simulink model "BLDCSpeedControl_EV_Layout_v2_backup_before_step3"  (R2024b)
settings: Solver=ode23t  StartTime=0.0  StopTime=0.3  FixedStep=Ts  MaxStep=5e-4  RelTol=1e-3  EnableMultiTasking=on
PreLoadFcn:
  | BLDCSpeedControlData;
PostLoadFcn:
  | % [EV_DAQ_V7_HOOK]
  | try; EV_DAQ_Builder_V7('LoadStop'); catch; end
InitFcn:
  | % [EV_DAQ_V7_HOOK]
  | try; EV_DAQ_Builder_V7('Overrides'); catch ME__daq; fprintf('[DAQ] Overrides error: %s\n', ME__daq.message); end
StartFcn:
  | % [EV_DAQ_V7_HOOK]
  | try; EV_DAQ_Builder_V7('AutoInit'); catch ME__daq; fprintf('[DAQ] Auto-init error: %s\n', ME__daq.message); end
StopFcn:
  | % [EV_DAQ_V7_HOOK]
  | try; EV_DAQ_Builder_V7('PostProcess'); catch ME__daq; fprintf('[DAQ] Post-process error: %s\n', ME__daq.message); end
undefined symbols (not defined in the file): battery_builder_rtmsupport, cells_parallel, cells_series, DiscIntNeverNeededParam, Emax, Emax_thr, emf_max_ev, gcbh, I_cont, I_peak, Ke_ph, Kii, Kiv, Kiw, Kpi, Kpv, Kpw, load_scale, p, r_wheel, rpm_ramp, rpm_ref, T_Ifilt, Ts, Tsc, Vdc, Vlim_min, wheel_mass
libraries: nesl_utility x17, fl_lib x17, ee_lib x6, eeDiscretePi x2, Batteries2_lib x1, SignalEditorBlockLib x1, eePwmGenerator x1, eeGeneralControl x1
(part 2 of 2)

== system BLDCSpeedControl_EV_Layout_v2_backup_before_step3/Speed//RPM Controller/Sign ==
  u : Inport
  Constant2 : Constant
  Constant3 : Constant  Value=-1
  Switch : Switch  SaturateOnIntegerOverflow=off  InputSameDT=off
  y : Outport
  wires:
  Constant3/1 -> Switch/3
  Constant2/1 -> Switch/1
  u/1 -> Switch/2
  Switch/1 -> y/1

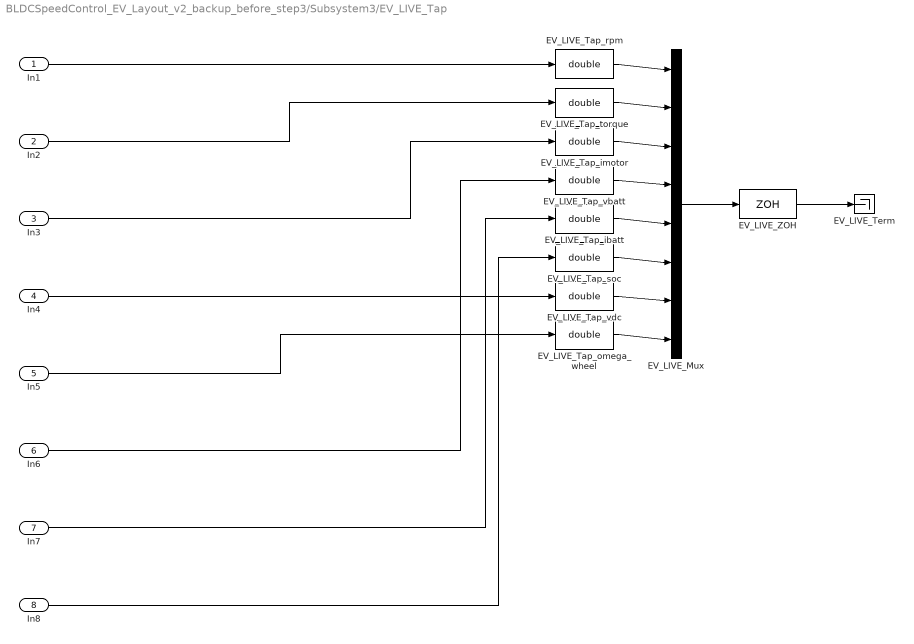
== system BLDCSpeedControl_EV_Layout_v2_backup_before_step3/Subsystem3/EV_LIVE_Tap ==
  In1 : Inport
  In2 : Inport  Port=2
  In3 : Inport  Port=3
  In4 : Inport  Port=4
  In5 : Inport  Port=5
  In6 : Inport  Port=6
  In7 : Inport  Port=7
  In8 : Inport  Port=8
  EV_LIVE_Mux : Mux  Inputs=8
  EV_LIVE_Tap_ibatt : DataTypeConversion  OutDataTypeStr=double
  EV_LIVE_Tap_imotor : DataTypeConversion  OutDataTypeStr=double
  EV_LIVE_Tap_omega_wheel : DataTypeConversion  OutDataTypeStr=double
  EV_LIVE_Tap_rpm : DataTypeConversion  OutDataTypeStr=double
  EV_LIVE_Tap_soc : DataTypeConversion  OutDataTypeStr=double
  EV_LIVE_Tap_torque : DataTypeConversion  OutDataTypeStr=double
  EV_LIVE_Tap_vbatt : DataTypeConversion  OutDataTypeStr=double
  EV_LIVE_Tap_vdc : DataTypeConversion  OutDataTypeStr=double
  EV_LIVE_Term : Terminator
  EV_LIVE_ZOH : ZeroOrderHold  SampleTime=0.1
  wires:
  EV_LIVE_Mux/1 -> EV_LIVE_ZOH/1
  EV_LIVE_Tap_rpm/1 -> EV_LIVE_Mux/1
  In5/1 -> EV_LIVE_Tap_omega_wheel/1
  EV_LIVE_Tap_imotor/1 -> EV_LIVE_Mux/3
  EV_LIVE_ZOH/1 -> EV_LIVE_Term/1
  EV_LIVE_Tap_torque/1 -> EV_LIVE_Mux/2
  EV_LIVE_Tap_ibatt/1 -> EV_LIVE_Mux/5
  In6/1 -> EV_LIVE_Tap_vbatt/1
  EV_LIVE_Tap_vbatt/1 -> EV_LIVE_Mux/4
  EV_LIVE_Tap_omega_wheel/1 -> EV_LIVE_Mux/8
  EV_LIVE_Tap_soc/1 -> EV_LIVE_Mux/6
  EV_LIVE_Tap_vdc/1 -> EV_LIVE_Mux/7
  In8/1 -> EV_LIVE_Tap_soc/1
  In1/1 -> EV_LIVE_Tap_rpm/1
  In2/1 -> EV_LIVE_Tap_torque/1
  In4/1 -> EV_LIVE_Tap_vdc/1
  In3/1 -> EV_LIVE_Tap_imotor/1
  In7/1 -> EV_LIVE_Tap_ibatt/1

== system BLDCSpeedControl_EV_Layout_v2_backup_before_step3/Subsystem3/Subsystem ==
  In1 : Inport
  In2 : Inport  Port=2
  In3 : Inport  Port=3
  In4 : Inport  Port=4
  In5 : Inport  Port=5
  In6 : Inport  Port=6
  In7 : Inport  Port=7

== system BLDCSpeedControl_EV_Layout_v2_backup_before_step3/Subsystem3/Subsystem1 ==
  In1 : Inport
  In2 : Inport  Port=2
  In3 : Inport  Port=3
  In4 : Inport  Port=4
  In5 : Inport  Port=5
  In6 : Inport  Port=6
  In7 : Inport  Port=7
  In8 : Inport  Port=8

== system BLDCSpeedControl_EV_Layout_v2_backup_before_step3/Subsystem3/Subsystem2 ==
  In1 : Inport
  In2 : Inport  Port=2
  In3 : Inport  Port=3
  In4 : Inport  Port=4
  In5 : Inport  Port=5
  In6 : Inport  Port=6
  In7 : Inport  Port=7
  In8 : Inport  Port=8

== system BLDCSpeedControl_EV_Layout_v2_backup_before_step3/Sensing w a/Hall sensor/Subsystem ==
  theta : Inport
  Trigonometric Function : Trigonometry  Operator=sincos
  Trigonometric Function2 : Trigonometry  Operator=atan2
  mech->elec : Gain  Gain=p
  rad->deg : Gain  Gain=180/pi  SaturateOnIntegerOverflow=on  OutDataTypeStr=Inherit: Same as input  ParamDataTypeStr=Inherit: Same as input
  deg : Outport  VectorParamsAs1DForOutWhenUnconnected=off
  wires:
  Trigonometric Function2/1 -> rad->deg/1
  Trigonometric Function/1 -> Trigonometric Function2/1
  theta/1 -> mech->elec/1
  rad->deg/1 -> deg/1
  Trigonometric Function/2 -> Trigonometric Function2/2
  mech->elec/1 -> Trigonometric Function/1

== system BLDCSpeedControl_EV_Layout_v2_backup_before_step3/Speed//RPM Controller/Commutation/Bit concatenate ==
  u : Inport
  Gain : Gain  Gain=[4 2 1]  Multiplication=Matrix(K*u)
  Sum of Elements : Sum  Inputs=+
  y : Outport  VectorParamsAs1DForOutWhenUnconnected=off
  wires:
  u/1 -> Gain/1
  Gain/1 -> Sum of Elements/1
  Sum of Elements/1 -> y/1
